simulink model "AFC_FFNN_trainlm_45_45_45_Nor_July_15"  (R2021a)
settings: Solver=ode15s  StartTime=0.0  StopTime=T  MaxStep=.01  RelTol=1e-3
undefined symbols (not defined in the file): AF_sensor_tol, fault_time, fuel_inj_tol, kappa_tol, MAF_sensor_tol, pump_tol, tau_ww_tol, x_gain, x_offset, y_gain, y_offset
libraries: neural x140
(part 1 of 6)
Description:
  | Modeling Engine Timing Using Triggered Subsystems
  | 
  | This example presents a model of a four-cylinder spark ignition engine
  | and demonstrates Simulink(R) capabilities to model an internal combustion
  | engine from the throttle to the crankshaft output. We used well-defined
  | physical principles supplemented, where appropriate, with empirical
  | relationships that describe the systems dynamic behavior without
  | introducing unnecessary complexity.
settings Model: SimulationMode=accelerator  ExtModeTrigMode=oneshot  ExtModeArmWhenConnect=off  ExtModeAutoUpdateStatusClock=off  Creator=The MathWorks Inc.  LastModifiedBy=deyun
settings SolverCC: ZeroCrossControl=DisableAll  AlgebraicLoopSolver=TrustRegion
settings DataIOCC: ExternalInput=[t__, u__]  LoadExternalInput=on  SaveFormat=StructureWithTime  SignalLogging=off  DSMLogging=off  ReturnWorkspaceOutputs=off
settings OptimizationCC: BlockReduction=off  BooleanDataType=off  LifeSpan=inf
settings DebuggingCC: SaveWithParameterizedLinksMsg=none  UnderspecifiedInitializationDetection=Classic  MergeDetectMultiDrivingBlocksExec=none  SignalResolutionControl=TryResolveAllWithWarning  ParameterPrecisionLossMsg=none  SFUnexpectedBacktrackingDiag=warning  SFNoUnconditionalDefaultTransitionDiag=warning  SFExecutionAtInitializationDiag=none  ArithmeticOperatorsInVariantConditions=warning
settings HardwareCC: ProdBitPerPointer=32  ProdBitPerSizeT=32  ProdBitPerPtrDiffT=32  ProdLargestAtomicFloat=None  ProdIntDivRoundTo=Undefined  ProdEndianess=Unspecified  ProdWordSize=32  ProdHWDeviceType=32-bit Generic  TargetBitPerLong=64  TargetBitPerPointer=64  TargetBitPerSizeT=64  TargetBitPerPtrDiffT=64  TargetLongLongMode=on  TargetIntDivRoundTo=Zero  TargetEndianess=LittleEndian  TargetWordSize=64  TargetHWDeviceType=MATLAB Host  ProdEqTarget=off
settings ModelReferenceCC: PropagateSignalLabelsOutOfModel=off
settings SFSimCC: SimUseLocalCustomCode=off  CustomCodeUndefinedFunction=UseInterfaceOnly
settings RTWCC: RTWUseLocalCustomCode=off
settings CodeAppCC: StateflowObjectComments=on
settings GRTTargetCC: TargetLangStandard=C89/C90 (ANSI)
settings ConfigComp: CovMetricSettings=d  CovSaveCumulativeToWorkspaceVar=on  CovSaveSingleToWorkspaceVar=on  CovExternalEMLEnable=off  CovBoundaryAbsTol=1.0e-5

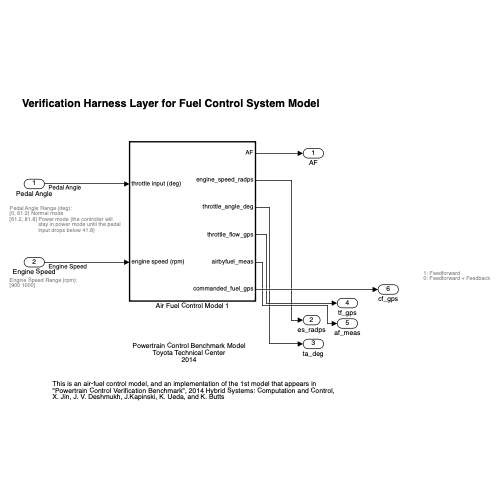
[thumbnail: Simulink's stored preview of the top-level diagram]
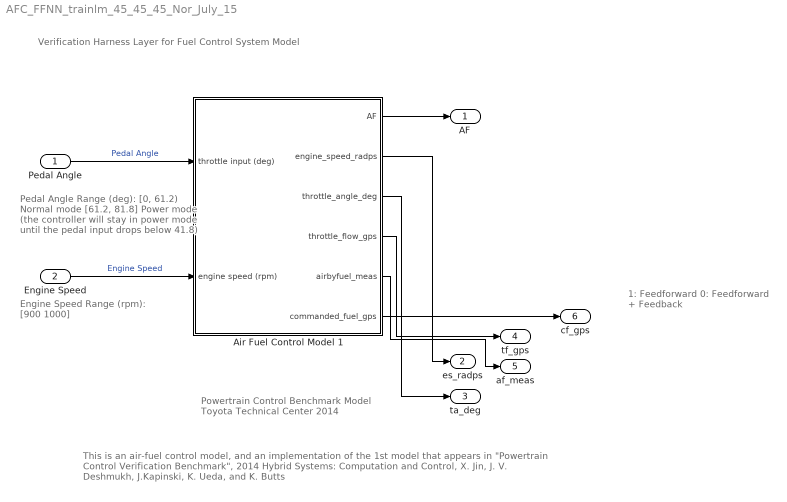
== system AFC_FFNN_trainlm_45_45_45_Nor_July_15 ==
  note: 1: Feedforward
      | 0: Feedforward + Feedback
  note: Pedal Angle Range (deg):
      | [0, 61.2) Normal mode
      | [61.2, 81.8] Power mode (the controller will
      |                    stay in power mode until the pedal
      |                    input drops below 41.8)
  note: This is an air-fuel control model, and an implementation of the 1st model that appears in
      | "Powertrain Control Verification Benchmark", 2014 Hybrid Systems: Computation and Control,
      | X. Jin, J. V. Deshmukh, J.Kapinski, K. Ueda, and K. Butts
  note: Engine Speed Range (rpm):
      | [900 1000]
  note: Powertrain Control Benchmark Model
      | Toyota Technical Center
      | 2014
  note: Verification Harness Layer for Fuel Control System Model
  Pedal Angle : Inport  Interpolate=off
  Engine Speed : Inport  Port=2  Interpolate=off
  Air Fuel Control Model 1 : Subsystem  Priority=1  TreatAsAtomicUnit=on
  AF : Outport  VectorParamsAs1DForOutWhenUnconnected=off
  es_radps : Outport  Port=2
  ta_deg : Outport  Port=3
  tf_gps : Outport  Port=4
  af_meas : Outport  Port=5
  cf_gps : Outport  Port=6
  wires:
  Air Fuel Control Model 1/1(AF) -> AF/1
  Pedal Angle/1 -> Air Fuel Control Model 1/1(throttle input (deg))  "Pedal Angle"
  Engine Speed/1 -> Air Fuel Control Model 1/2(engine speed (rpm))  "Engine Speed"
  Air Fuel Control Model 1/2(engine_speed_radps) -> es_radps/1
  Air Fuel Control Model 1/3(throttle_angle_deg) -> ta_deg/1
  Air Fuel Control Model 1/4(throttle_flow_gps) -> tf_gps/1
  Air Fuel Control Model 1/5(airbyfuel_meas) -> af_meas/1
  Air Fuel Control Model 1/6(commanded_fuel_gps) -> cf_gps/1

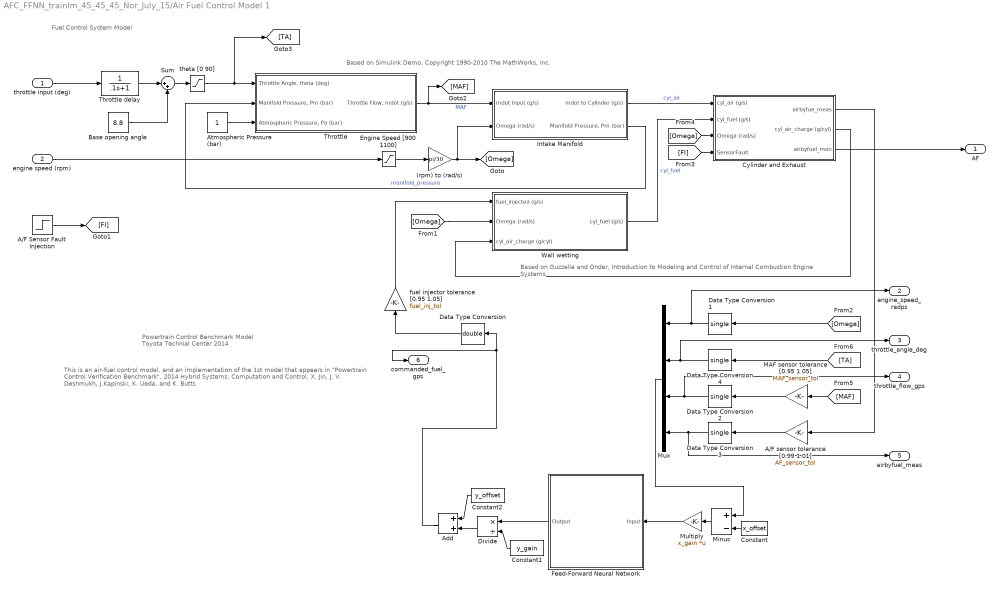
== system AFC_FFNN_trainlm_45_45_45_Nor_July_15/Air Fuel Control Model 1 ==
  note: Based on Simulink Demo, Copyright 1990-2010 The MathWorks, Inc.
  note: Based on Guzzella and Onder, Introduction to Modeling and Control of Internal Combustion Engine Systems
  note: Fuel Control System Model
  note: This is an air-fuel control model, and an implementation of the 1st model that appears in
      | "Powertrain Control Verification Benchmark", 2014 Hybrid Systems: Computation and Control,
      | X. Jin, J. V. Deshmukh, J.Kapinski, K. Ueda, and K. Butts
  note: Powertrain Control Benchmark Model
      | Toyota Technial Center
      | 2014
  throttle input (deg) : Inport  Description=[0, 81.2]
      settings: AttributesFormatString=%<Description>
  engine speed (rpm) : Inport  Description=[900,1100]  Port=2
      settings: AttributesFormatString=%<Description>
  (rpm) to (rad/s) : Gain  Gain=pi/30
  A/F Sensor Fault Injection : Step  Time=fault_time  SampleTime=0
      settings: AttributesFormatString=1: Failure\n0: Normal
  A/F sensor tolerance [0.99 1.01] : Gain  Gain=AF_sensor_tol
  Add : Sum
  Atmospheric Pressure (bar) : Constant
  Base opening angle : Constant  Value=8.8
  Constant : Constant  Value=x_offset
  Constant1 : Constant  Value=y_gain
  Constant2 : Constant  Value=y_offset
  Cylinder and Exhaust : Subsystem
  Data Type Conversion : DataTypeConversion  OutDataTypeStr=double
  Data Type Conversion{1..4} (4 alike) : DataTypeConversion  OutDataTypeStr=single
  Divide : Product  Inputs=*/
  Engine Speed [900 1100] : Saturate  UpperLimit=1100  LowerLimit=900
  Feed-Forward Neural Network : Subsystem
      mask help: Feed-Forward Neural Network
      mask Display: e = 0.06;c1 = [120 150 230]/255;c2 = ([120 150 230]+0)/383;c3 = ([120 150 230]+128)/383;patch([0 1 1 0],[0 0 1 1],c1);patch([0 1 1 1-e 1-e 0+e],[0 0 1 1-e 0+e 0+e],c2);patch([0 0 1 1-e 0+e 0+e],[0 1 1 1-e 1-e 0+e],c3);plot([0 1 1 0 0],[0 0 1 1 0]);fprintf('NNET');port_label('input',1,' Input');port_label('output',1,'Output ');
  Intake Manifold : Subsystem
  MAF sensor tolerance [0.95 1.05] : Gain  Gain=MAF_sensor_tol
  Minus : Sum  Inputs=+-
  Multiply : Gain  Gain=x_gain  Multiplication=Matrix(K*u)
  Mux : Mux
  Sum : Sum  Inputs=|++
  Throttle : Subsystem
  Throttle delay : TransferFcn  Denominator=[.1 1]
  Wall wetting : Subsystem
  fuel injector tolerance [0.95 1.05] : Gain  Gain=fuel_inj_tol
  theta [0 90] : Saturate  UpperLimit=90  LowerLimit=0
  AF : Outport  VectorParamsAs1DForOutWhenUnconnected=off
  engine_speed_radps : Outport  Port=2
  throttle_angle_deg : Outport  Port=3
  throttle_flow_gps : Outport  Port=4
  airbyfuel_meas : Outport  Port=5
  commanded_fuel_gps : Outport  Port=6
  wires:
  (rpm) to (rad/s)/1 -> [Omega], Intake Manifold/2(Omega (rad/s))
  Data Type Conversion/1 -> fuel injector tolerance [0.95 1.05]/1
  theta [0 90]/1 -> Throttle/1("Throttle Angle, theta (deg)"), [TA]
  Engine Speed [900 1100]/1 -> (rpm) to (rad/s)/1
  Cylinder and Exhaust/3("airbyfuel_mon ") -> AF/1
  A/F sensor tolerance [0.99 1.01]/1 -> Data Type Conversion3/1
  [MAF] -> MAF sensor tolerance [0.95 1.05]/1
  Cylinder and Exhaust/1(airbyfue_meas) -> A/F sensor tolerance [0.99 1.01]/1
  Throttle/1("Throttle Flow, mdot (g/s)") -> [MAF], Intake Manifold/1(mdot Input (g/s))  "MAF"
  Intake Manifold/2("Manifold Pressure, Pm (bar)") -> Throttle/2("Manifold Pressure, Pm (bar)")  "manifold_pressure"
  Atmospheric Pressure (bar)/1 -> Throttle/3("Atmospheric Pressure, Pa (bar) ")
  Wall wetting/1(cyl_fuel (g/s)) -> Cylinder and Exhaust/2(cyl_fuel (g/s))  "cyl_fuel"
  Intake Manifold/1(mdot to Cylinder (g/s)) -> Cylinder and Exhaust/1(cyl_air (g/s))  "cyl_air"
  [Omega] -> Cylinder and Exhaust/3(Omega (rad/s))
  [Omega] -> Wall wetting/2(Omega (rad/s))
  Cylinder and Exhaust/2(cyl_air_charge (g/cyl)) -> Wall wetting/3(cyl_air_charge (g/cyl))
  [Omega] -> Data Type Conversion1/1
  fuel injector tolerance [0.95 1.05]/1 -> Wall wetting/1(fuel_injected (g/s))
  MAF sensor tolerance [0.95 1.05]/1 -> Data Type Conversion2/1
  Add/1 -> Data Type Conversion/1, commanded_fuel_gps/1
  A/F Sensor Fault Injection/1 -> [FI]
  [FI] -> Cylinder and Exhaust/4(SensorFault)
  [TA] -> Data Type Conversion4/1
  throttle input (deg)/1 -> Throttle delay/1
  engine speed (rpm)/1 -> Engine Speed [900 1100]/1
  Throttle delay/1 -> Sum/1
  Base opening angle/1 -> Sum/2
  Sum/1 -> theta [0 90]/1
  Data Type Conversion3/1 -> airbyfuel_meas/1, Mux/4
  Data Type Conversion4/1 -> Mux/2, throttle_angle_deg/1
  Data Type Conversion2/1 -> Mux/3, throttle_flow_gps/1
  Data Type Conversion1/1 -> Mux/1, engine_speed_radps/1
  Multiply/1 -> Feed-Forward Neural Network/1(Input)
  Constant/1 -> Minus/2
  Mux/1 -> Minus/1
  Minus/1 -> Multiply/1
  Constant2/1 -> Add/1
  Feed-Forward Neural Network/1(Output) -> Divide/1
  Constant1/1 -> Divide/2
  Divide/1 -> Add/2

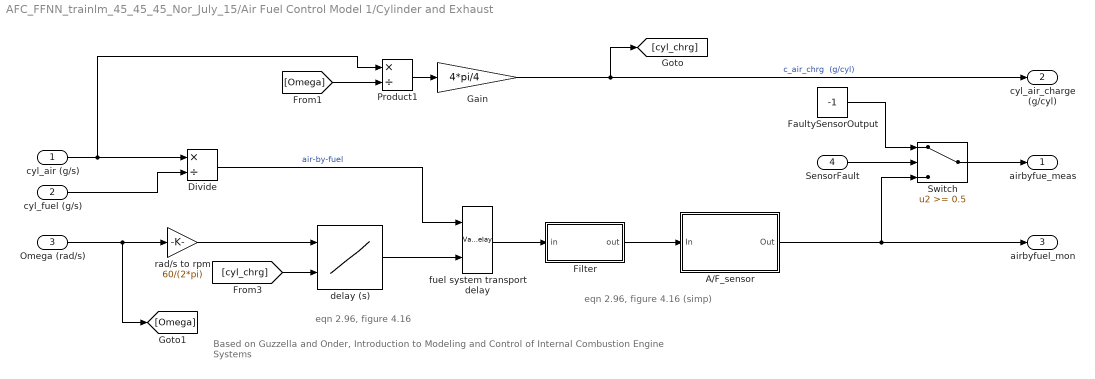
== system AFC_FFNN_trainlm_45_45_45_Nor_July_15/Air Fuel Control Model 1/Cylinder and Exhaust ==
  note: Based on Guzzella and Onder, Introduction to Modeling and Control of Internal Combustion Engine Systems
  note: eqn 2.96, figure 4.16
  note: eqn 2.96, figure 4.16 (simp)
  cyl_air (g/s) : Inport
  cyl_fuel (g/s) : Inport  Port=2
  Omega (rad/s) : Inport  Port=3
  SensorFault : Inport  Port=4
  A/F_sensor : Subsystem
  Divide : Product  Inputs=*/
  FaultySensorOutput : Constant  Value=-1
  Filter : Subsystem
  Gain : Gain  Gain=4*pi/4
  Product1 : Product  Inputs=*/  RndMeth=Zero
  Switch : Switch  Threshold=0.5
  delay (s) : Lookup_n-D  BreakpointsForDimension1=[800,1000,1500,2000,3000]  BreakpointsForDimension2=[0.05,0.15,0.2,0.25]  Table=reshape([0.8,0.6,0.4,0.3,0.2,0.4,0.3,0.2,0.2,0.2,0.3,0.25,0.2,0.2,0.2,0.25,0.2,0.2,0.2,0.2],5,4)  UseLastTableValue=on  RndMeth=Simplest  InputSameDT=on
      settings: InputPortMap=u0,u1
  fuel system transport delay : VariableTransportDelay  VariableDelayType=Variable transport delay  MaximumDelay=10  InitialOutput=14.7  MaximumPoints=20480
  rad/s to rpm : Gain  Gain=60/(2*pi)
  airbyfue_meas : Outport  VectorParamsAs1DForOutWhenUnconnected=off
  cyl_air_charge (g/cyl) : Outport  Port=2  VectorParamsAs1DForOutWhenUnconnected=off
  "airbyfuel_mon " : Outport  Port=3  VectorParamsAs1DForOutWhenUnconnected=off
  wires:
  cyl_air (g/s)/1 -> Divide/1, Product1/1
  [Omega] -> Product1/2
  Product1/1 -> Gain/1
  Gain/1 -> [cyl_chrg], cyl_air_charge (g/cyl)/1  "c_air_chrg  (g/cyl)"
  [cyl_chrg] -> delay (s)/2
  cyl_fuel (g/s)/1 -> Divide/2
  Omega (rad/s)/1 -> [Omega], rad/s to rpm/1
  rad/s to rpm/1 -> delay (s)/1
  delay (s)/1 -> fuel system transport delay/2
  fuel system transport delay/1 -> Filter/1(in)
  Switch/1 -> airbyfue_meas/1
  Divide/1 -> fuel system transport delay/1  "air-by-fuel"
  Filter/1(out) -> A/F_sensor/1(In)
  FaultySensorOutput/1 -> Switch/1
  SensorFault/1 -> Switch/2
  A/F_sensor/1(Out) -> Switch/3, "airbyfuel_mon "/1

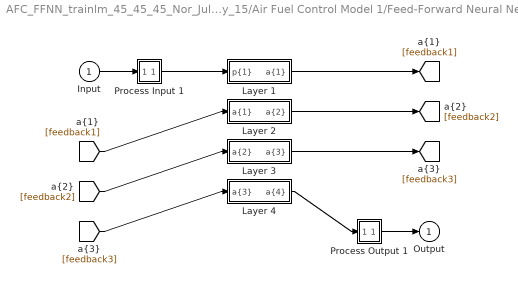
== system AFC_FFNN_trainlm_45_45_45_Nor_July_15/Air Fuel Control Model 1/Feed-Forward Neural Network ==
  Input : Inport  PortDimensions=4
      mask Display: e = 0.06;c1 = [120 230 180]/255;c2 = ([120 230 180]+0)/(256+128);c3 = ([120 230 180]+128)/(256+128);patch([0 1 1 0],[0 0 1 1],c1);patch([0 1 1 1-e 1-e 0+e],[0 0 1 1-e 0+e 0+e],c2);patch([0 0 1 1-e 0+e 0+e],[0 1 1 1-e 1-e 0+e],c3);plot([0 1 1 0 0],[0 0 1 1 0]);
  Layer 1 : Subsystem
      mask Display: e = 0.06;c1 = [120 150 230]/255;c2 = ([120 150 230]+0)/383;c3 = ([120 150 230]+128)/383;patch([0 1 1 0],[0 0 1 1],c1);patch([0 1 1 1-e 1-e 0+e],[0 0 1 1-e 0+e 0+e],c2);patch([0 0 1 1-e 0+e 0+e],[0 1 1 1-e 1-e 0+e],c3);plot([0 1 1 0 0],[0 0 1 1 0]);
  Layer 2 : Subsystem
      mask Display: e = 0.06;c1 = [120 150 230]/255;c2 = ([120 150 230]+0)/383;c3 = ([120 150 230]+128)/383;patch([0 1 1 0],[0 0 1 1],c1);patch([0 1 1 1-e 1-e 0+e],[0 0 1 1-e 0+e 0+e],c2);patch([0 0 1 1-e 0+e 0+e],[0 1 1 1-e 1-e 0+e],c3);plot([0 1 1 0 0],[0 0 1 1 0]);
  Layer 3 : Subsystem
      mask Display: e = 0.06;c1 = [120 150 230]/255;c2 = ([120 150 230]+0)/383;c3 = ([120 150 230]+128)/383;patch([0 1 1 0],[0 0 1 1],c1);patch([0 1 1 1-e 1-e 0+e],[0 0 1 1-e 0+e 0+e],c2);patch([0 0 1 1-e 0+e 0+e],[0 1 1 1-e 1-e 0+e],c3);plot([0 1 1 0 0],[0 0 1 1 0]);
  Layer 4 : Subsystem
      mask Display: e = 0.06;c1 = [120 150 230]/255;c2 = ([120 150 230]+0)/383;c3 = ([120 150 230]+128)/383;patch([0 1 1 0],[0 0 1 1],c1);patch([0 1 1 1-e 1-e 0+e],[0 0 1 1-e 0+e 0+e],c2);patch([0 0 1 1-e 0+e 0+e],[0 1 1 1-e 1-e 0+e],c3);plot([0 1 1 0 0],[0 0 1 1 0]);
  Process Input 1 : Subsystem
      mask Display: e = 0.06;c1 = [120 150 230]/255;c2 = ([120 150 230]+0)/383;c3 = ([120 150 230]+128)/383;patch([0 1 1 0],[0 0 1 1],c1);patch([0 1 1 1-e 1-e 0+e],[0 0 1 1-e 0+e 0+e],c2);patch([0 0 1 1-e 0+e 0+e],[0 1 1 1-e 1-e 0+e],c3);plot([0 1 1 0 0],[0 0 1 1 0]);
  Process Output 1 : Subsystem
      mask Display: e = 0.06;c1 = [120 150 230]/255;c2 = ([120 150 230]+0)/383;c3 = ([120 150 230]+128)/383;patch([0 1 1 0],[0 0 1 1],c1);patch([0 1 1 1-e 1-e 0+e],[0 0 1 1-e 0+e 0+e],c2);patch([0 0 1 1-e 0+e 0+e],[0 1 1 1-e 1-e 0+e],c3);plot([0 1 1 0 0],[0 0 1 1 0]);
  Output : Outport  InitialOutput=0
      mask Display: e = 0.06;c1 = [120 230 180]/255;c2 = ([120 230 180]+0)/(256+128);c3 = ([120 230 180]+128)/(256+128);patch([0 1 1 0],[0 0 1 1],c1);patch([0 1 1 1-e 1-e 0+e],[0 0 1 1-e 0+e 0+e],c2);patch([0 0 1 1-e 0+e 0+e],[0 1 1 1-e 1-e 0+e],c3);plot([0 1 1 0 0],[0 0 1 1 0]);
  wires:
  Layer 4/1("a{4}") -> Process Output 1/1(a)
  [feedback3] -> Layer 4/1("a{3} ")
  Layer 3/1("a{3}") -> [feedback3]
  [feedback2] -> Layer 3/1("a{2} ")
  Layer 2/1("a{2}") -> [feedback2]
  [feedback1] -> Layer 2/1("a{1} ")
  Layer 1/1("a{1}") -> [feedback1]
  Process Input 1/1(p) -> Layer 1/1("p{1}")
  Process Output 1/1(y) -> Output/1
  Input/1 -> Process Input 1/1(x)

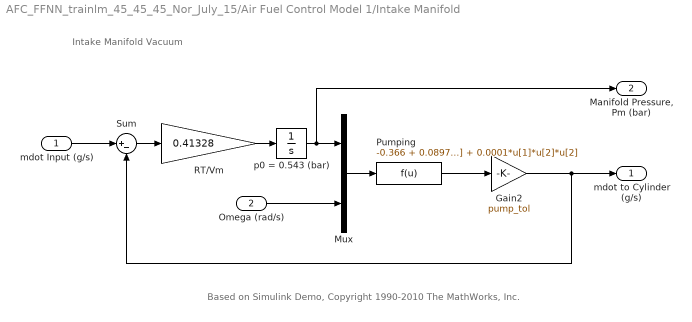
== system AFC_FFNN_trainlm_45_45_45_Nor_July_15/Air Fuel Control Model 1/Intake Manifold ==
  note: Intake Manifold Vacuum
  note: Based on Simulink Demo, Copyright 1990-2010 The MathWorks, Inc.
  mdot Input (g/s) : Inport
  Omega (rad/s) : Inport  Port=2
  Gain2 : Gain  Gain=pump_tol  ParamDataTypeStr=single  OutDataTypeStr=Inherit: Inherit via back propagation  RndMeth=Simplest  SaturateOnIntegerOverflow=on
      settings: AttributesFormatString=pumping tolerance [0.9 1.1]
  Mux : Mux  Inputs=2
  Pumping : Fcn  Expr=-0.366 + 0.08979*u[1]*u[2] - 0.0337*u[2]*u[1]*u[1] + 0.0001*u[1]*u[2]*u[2]
  RT/Vm : Gain  Gain=0.41328  SaturateOnIntegerOverflow=on  OutDataTypeStr=Inherit: Same as input  ParamDataTypeStr=Inherit: Same as input
  Sum : Sum  Inputs=|+-  InputSameDT=on  SaturateOnIntegerOverflow=on  OutDataTypeStr=Inherit: Same as first input
  p0 = 0.543 (bar) : Integrator  InitialCondition=0.982
  mdot to Cylinder (g/s) : Outport  InitialOutput=0  VectorParamsAs1DForOutWhenUnconnected=off
  "Manifold Pressure, Pm (bar)" : Outport  Port=2  InitialOutput=0  VectorParamsAs1DForOutWhenUnconnected=off
  wires:
  mdot Input (g/s)/1 -> Sum/1
  RT/Vm/1 -> p0 = 0.543 (bar)/1
  Omega (rad/s)/1 -> Mux/2
  Mux/1 -> Pumping/1
  p0 = 0.543 (bar)/1 -> Mux/1, "Manifold Pressure, Pm (bar)"/1
  Sum/1 -> RT/Vm/1
  Pumping/1 -> Gain2/1
  Gain2/1 -> Sum/2, mdot to Cylinder (g/s)/1

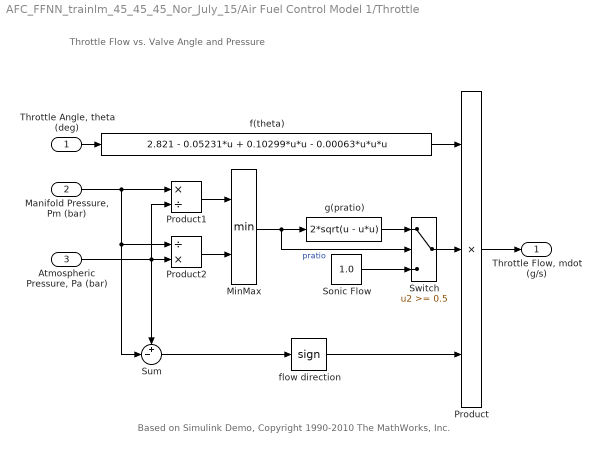
== system AFC_FFNN_trainlm_45_45_45_Nor_July_15/Air Fuel Control Model 1/Throttle ==
  note: Throttle Flow vs. Valve Angle and Pressure
  note: Based on Simulink Demo, Copyright 1990-2010 The MathWorks, Inc.
  "Throttle Angle, theta (deg)" : Inport
  "Manifold Pressure, Pm (bar)" : Inport  Port=2
  "Atmospheric Pressure, Pa (bar) " : Inport  Port=3
  MinMax : MinMax  Inputs=2  InputSameDT=on  SaturateOnIntegerOverflow=on
  Product : Product  Inputs=3  InputSameDT=on  RndMeth=Zero  SaturateOnIntegerOverflow=on  OutDataTypeStr=Inherit: Same as first input
  Product1 : Product  Inputs=*/  InputSameDT=on  RndMeth=Zero  SaturateOnIntegerOverflow=on  OutDataTypeStr=Inherit: Same as first input
  Product2 : Product  Inputs=/*  InputSameDT=on  RndMeth=Zero  SaturateOnIntegerOverflow=on  OutDataTypeStr=Inherit: Same as first input
  "Sonic Flow " : Constant  Value=1.0
  Sum : Sum  Inputs=+-|  InputSameDT=on  SaturateOnIntegerOverflow=on  OutDataTypeStr=Inherit: Same as first input
  Switch : Switch  Threshold=0.5  SaturateOnIntegerOverflow=on  InputSameDT=on
  f(theta) : Fcn  Expr=2.821 - 0.05231*u + 0.10299*u*u - 0.00063*u*u*u
  flow direction : Signum
  g(pratio) : Fcn  Expr=2*sqrt(u - u*u)
  "Throttle Flow, mdot (g/s)" : Outport  InitialOutput=0  VectorParamsAs1DForOutWhenUnconnected=off
  wires:
  "Manifold Pressure, Pm (bar)"/1 -> Sum/2, Product2/1, Product1/1
  Product2/1 -> MinMax/2
  Product1/1 -> MinMax/1
  "Atmospheric Pressure, Pa (bar) "/1 -> Sum/1, Product2/2, Product1/2
  g(pratio)/1 -> Switch/1
  "Sonic Flow "/1 -> Switch/3
  Switch/1 -> Product/2
  flow direction/1 -> Product/3
  Sum/1 -> flow direction/1
  MinMax/1 -> g(pratio)/1, Switch/2  "pratio"
  "Throttle Angle, theta (deg)"/1 -> f(theta)/1
  Product/1 -> "Throttle Flow, mdot (g/s)"/1
  f(theta)/1 -> Product/1

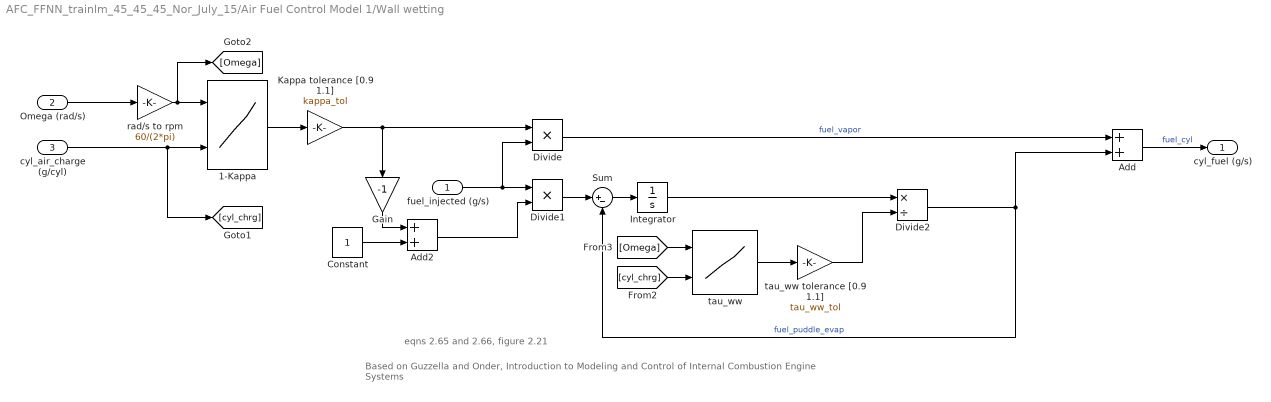
== system AFC_FFNN_trainlm_45_45_45_Nor_July_15/Air Fuel Control Model 1/Wall wetting ==
  note: Based on Guzzella and Onder, Introduction to Modeling and Control of Internal Combustion Engine Systems
  note: eqns 2.65 and 2.66, figure 2.21
  fuel_injected (g/s) : Inport
  Omega (rad/s) : Inport  Port=2
  cyl_air_charge (g/cyl) : Inport  Port=3
  1-Kappa : Lookup_n-D  BreakpointsForDimension1=[1000,1500,2000,2500,3000]  BreakpointsForDimension2=[.1,.2,.3,.4]  Table=reshape([0.8,.7,.7,.8,.9,.7,.66,.65,.73,.85,.66,.66,.63,.66,.8,.6,.6,.6,.6,.7],5,4)  UseLastTableValue=on  RndMeth=Simplest  InputSameDT=on
      settings: InputPortMap=u0,u1
  Add : Sum
  Add2 : Sum
  Constant : Constant
  Divide : Product  Inputs=**
  Divide1 : Product  Inputs=**
  Divide2 : Product  Inputs=*/
  Gain : Gain  Gain=-1
  Integrator : Integrator  InitialCondition=.0112
  Kappa tolerance [0.9 1.1] : Gain  Gain=kappa_tol
  Sum : Sum  Inputs=|+-
  rad/s to rpm : Gain  Gain=60/(2*pi)
  tau_ww : Lookup_n-D  BreakpointsForDimension1=[1000,1500,2000,2500,3000]  BreakpointsForDimension2=[0.1,0.2,0.3,0.4]  Table=reshape([.4,.3,.35,.3,.2,.22,.22,.4,.35,.5,.20,.22,.5,.4,.35,.35,.3,.45,.5,.4],5,4)  UseLastTableValue=on  RndMeth=Simplest  InputSameDT=on
      settings: InputPortMap=u0,u1
  tau_ww tolerance [0.9 1.1] : Gain  Gain=tau_ww_tol
  cyl_fuel (g/s) : Outport  VectorParamsAs1DForOutWhenUnconnected=off
  wires:
  1-Kappa/1 -> Kappa tolerance [0.9 1.1]/1
  fuel_injected (g/s)/1 -> Divide/2, Divide1/1
  Divide/1 -> Add/1  "fuel_vapor"
  Add/1 -> cyl_fuel (g/s)/1  "fuel_cyl"
  Integrator/1 -> Divide2/1
  Divide1/1 -> Sum/1
  Sum/1 -> Integrator/1
  Divide2/1 -> Add/2, Sum/2  "fuel_puddle_evap"
  Add2/1 -> Divide1/2
  cyl_air_charge (g/cyl)/1 -> 1-Kappa/2, [cyl_chrg]
  [cyl_chrg] -> tau_ww/2
  tau_ww/1 -> tau_ww tolerance [0.9 1.1]/1
  Gain/1 -> Add2/1
  Constant/1 -> Add2/2
  rad/s to rpm/1 -> [Omega], 1-Kappa/1
  Omega (rad/s)/1 -> rad/s to rpm/1
  Kappa tolerance [0.9 1.1]/1 -> Divide/1, Gain/1
  tau_ww tolerance [0.9 1.1]/1 -> Divide2/2
  [Omega] -> tau_ww/1

== system AFC_FFNN_trainlm_45_45_45_Nor_July_15/Air Fuel Control Model 1/Cylinder and Exhaust/A//F_sensor ==
  In : Inport
  A/F_sensor : Gain  OutDataTypeStr=double
  Filter : Subsystem
  Out : Outport  VectorParamsAs1DForOutWhenUnconnected=off
  wires:
  A/F_sensor/1 -> Out/1
  In/1 -> Filter/1(In)
  Filter/1(Out) -> A/F_sensor/1

== system AFC_FFNN_trainlm_45_45_45_Nor_July_15/Air Fuel Control Model 1/Cylinder and Exhaust/Filter ==
  in : Inport
  Gain1 : Gain  Gain=10
  Integrator : Integrator  InitialCondition=14.7
  Sum : Sum  Inputs=|+-
  out : Outport  VectorParamsAs1DForOutWhenUnconnected=off
  wires:
  Integrator/1 -> out/1, Sum/2
  in/1 -> Sum/1
  Gain1/1 -> Integrator/1
  Sum/1 -> Gain1/1

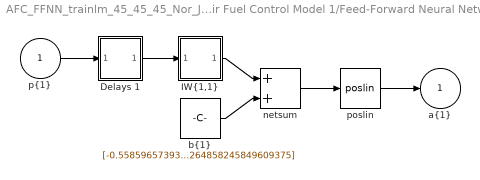
== system AFC_FFNN_trainlm_45_45_45_Nor_July_15/Air Fuel Control Model 1/Feed-Forward Neural Network/Layer 1 ==
  "p{1}" : Inport  PortDimensions=4
      mask Display: e = 0.06;c1 = [120 230 180]/255;c2 = ([120 230 180]+0)/(256+128);c3 = ([120 230 180]+128)/(256+128);patch([0 1 1 0],[0 0 1 1],c1);patch([0 1 1 1-e 1-e 0+e],[0 0 1 1-e 0+e 0+e],c2);patch([0 0 1 1-e 0+e 0+e],[0 1 1 1-e 1-e 0+e],c3);plot([0 1 1 0 0],[0 0 1 1 0]);
  Delays 1 : Subsystem
      mask Display: e = 0.06;c1 = [120 150 230]/255;c2 = ([120 150 230]+0)/383;c3 = ([120 150 230]+128)/383;patch([0 1 1 0],[0 0 1 1],c1);patch([0 1 1 1-e 1-e 0+e],[0 0 1 1-e 0+e 0+e],c2);patch([0 0 1 1-e 0+e 0+e],[0 1 1 1-e 1-e 0+e],c3);plot([0 1 1 0 0],[0 0 1 1 0]);disp('0');
  "IW{1,1}" : Subsystem
      mask Display: e = 0.06;c1 = [120 150 230]/255;c2 = ([120 150 230]+0)/383;c3 = ([120 150 230]+128)/383;patch([0 1 1 0],[0 0 1 1],c1);patch([0 1 1 1-e 1-e 0+e],[0 0 1 1-e 0+e 0+e],c2);patch([0 0 1 1-e 0+e 0+e],[0 1 1 1-e 1-e 0+e],c3);plot([0 1 1 0 0],[0 0 1 1 0]);disp('W');
  "b{1}" : Constant  Value=[-0.5585965739320057910077821361483074724674224853515625;-0.77112950387139012065063070622272789478302001953125;0.22894666757716020111246280066552571952342987060546875;-0.305047379583083699827739110332913696765899658203125;-0.69451441467543661989481051932671107351779937744140625;0.39214635280524723359718564097420312464237213134765625;-0.1555721937487436756786252090023481287062168121337890625;0.274827394729951490770503141902736388146877288818359375;0.277365245819692296525005303919897414743900299072265625;-0.1524186026109950187201746985010686330497264862060546875;-0.0018307247949869154268753845826722681522369384765625;0.58822997451524916545650967236724682152271270751953125;0.55084837701463318371253308214363642036914825439453125;0.314130170445041712046219117837608791887760162353515625;-0.07693509824360840465562461076842737384140491485595703125;-0.851136421274869547914931899867951869964599609375;0.362298342175110754670441792768542654812335968017578125;0.21255578744349323816464902847656048834323883056640625;-0.3824877228684744334685774447279982268810272216796875;-0.6749591132024963524571603556978516280651092529296875;-0.63890547966722144312967657242552377283573150634765625;-0.149732930796697971675968119598110206425189971923828125;-0.933207190422134402751908055506646633148193359375;0.10402318613955320592001640989110455848276615142822265625;0.829936502547987675626472992007620632648468017578125;-0.737888972575629242811601216089911758899688720703125;0.21732415928306558772220569153432734310626983642578125;-0.1580532967861125737130123525275848805904388427734375;-1.288298758066100280217369800084270536899566650390625;-0.9481540190806569956549765265663154423236846923828125;0.942806016112406108931054404820315539836883544921875;-0.439159443551665196192601570146507583558559417724609375;0.276425093592411907916783775363001041114330291748046875;0.485464567417084047473707641984219662845134735107421875;0.295746825087029263645632681800634600222110748291015625;-0.8382271786519968070905406420934014022350311279296875;-0.1591390063283328881738043492077849805355072021484375;-0.7823304156725818803153060798649676144123077392578125;0.2224216466664273028630560702367802150547504425048828125;0.75721224172485557257772370576276443898677825927734375;-0.26127862544034818892413341018254868686199188232421875;0.1681522472301393289484394699684344232082366943359375;0.00998894613673773079653983586467802524566650390625;-0.6614665456480552929718896848498843610286712646484375;-0.838290046288482582070855642086826264858245849609375]
      mask Display: e = 0.06;c1 = [120 150 230]/255;c2 = ([120 150 230]+0)/383;c3 = ([120 150 230]+128)/383;patch([0 1 1 0],[0 0 1 1],c1);patch([0 1 1 1-e 1-e 0+e],[0 0 1 1-e 0+e 0+e],c2);patch([0 0 1 1-e 0+e 0+e],[0 1 1 1-e 1-e 0+e],c3);plot([0 1 1 0 0],[0 0 1 1 0]);disp('b');
  netsum : Sum  Inputs=2  InputSameDT=on  SaturateOnIntegerOverflow=on  OutDataTypeStr=Inherit: Same as first input
      mask Display: e = 0.06;c1 = [120 150 230]/255;c2 = ([120 150 230]+0)/383;c3 = ([120 150 230]+128)/383;patch([0 1 1 0],[0 0 1 1],c1);patch([0 1 1 1-e 1-e 0+e],[0 0 1 1-e 0+e 0+e],c2);patch([0 0 1 1-e 0+e 0+e],[0 1 1 1-e 1-e 0+e],c3);plot([0 1 1 0 0],[0 0 1 1 0]);disp('+');
  poslin : neural/Transfer Functions/poslin
  "a{1}" : Outport  InitialOutput=[0;0;0;0;0;0;0;0;0;0;0;0;0;0;0;0;0;0;0;0;0;0;0;0;0;0;0;0;0;0;0;0;0;0;0;0;0;0;0;0;0;0;0;0;0]
      mask Display: e = 0.06;c1 = [120 230 180]/255;c2 = ([120 230 180]+0)/(256+128);c3 = ([120 230 180]+128)/(256+128);patch([0 1 1 0],[0 0 1 1],c1);patch([0 1 1 1-e 1-e 0+e],[0 0 1 1-e 0+e 0+e],c2);patch([0 0 1 1-e 0+e 0+e],[0 1 1 1-e 1-e 0+e],c3);plot([0 1 1 0 0],[0 0 1 1 0]);
  wires:
  poslin/1 -> "a{1}"/1
  netsum/1 -> poslin/1
  "b{1}"/1 -> netsum/2
  "IW{1,1}"/1("iz{1,1}") -> netsum/1
  Delays 1/1("pd{1,1}") -> "IW{1,1}"/1("pd{1,1}")
  "p{1}"/1 -> Delays 1/1("p{1}")

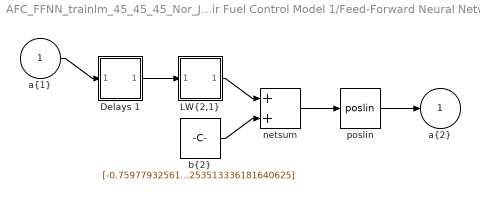
== system AFC_FFNN_trainlm_45_45_45_Nor_July_15/Air Fuel Control Model 1/Feed-Forward Neural Network/Layer 2 ==
  "a{1} " : Inport  PortDimensions=45
      mask Display: e = 0.06;c1 = [120 230 180]/255;c2 = ([120 230 180]+0)/(256+128);c3 = ([120 230 180]+128)/(256+128);patch([0 1 1 0],[0 0 1 1],c1);patch([0 1 1 1-e 1-e 0+e],[0 0 1 1-e 0+e 0+e],c2);patch([0 0 1 1-e 0+e 0+e],[0 1 1 1-e 1-e 0+e],c3);plot([0 1 1 0 0],[0 0 1 1 0]);
  Delays 1 : Subsystem
      mask Display: e = 0.06;c1 = [120 150 230]/255;c2 = ([120 150 230]+0)/383;c3 = ([120 150 230]+128)/383;patch([0 1 1 0],[0 0 1 1],c1);patch([0 1 1 1-e 1-e 0+e],[0 0 1 1-e 0+e 0+e],c2);patch([0 0 1 1-e 0+e 0+e],[0 1 1 1-e 1-e 0+e],c3);plot([0 1 1 0 0],[0 0 1 1 0]);disp('0');
  "LW{2,1}" : Subsystem
      mask Display: e = 0.06;c1 = [120 150 230]/255;c2 = ([120 150 230]+0)/383;c3 = ([120 150 230]+128)/383;patch([0 1 1 0],[0 0 1 1],c1);patch([0 1 1 1-e 1-e 0+e],[0 0 1 1-e 0+e 0+e],c2);patch([0 0 1 1-e 0+e 0+e],[0 1 1 1-e 1-e 0+e],c3);plot([0 1 1 0 0],[0 0 1 1 0]);disp('W');
  "b{2}" : Constant  Value=[-0.759779325613544553874589837505482137203216552734375;0.6965202526642186864336281360010616481304168701171875;-0.861179161880855748023577689309604465961456298828125;0.279069361418990080636604034225456416606903076171875;0.7788995695670519747721982639632187783718109130859375;0.72059847295826762181292224340722896158695220947265625;0.56823299771985691375419946780311875045299530029296875;-0.814016852489903186551600811071693897247314453125;-0.25020043213131148984729179574060253798961639404296875;0.3676809986895264170669861414353363215923309326171875;-0.5664709440966280151741329973447136580944061279296875;0.02629409189089770837455262153525836765766143798828125;-0.54936854809591240123012312324135564267635345458984375;-0.133862432529689490134927609688020311295986175537109375;-0.81332808228198449906898304107016883790493011474609375;-0.75199519420301730310285392988589592278003692626953125;-1.0530530335707963818236976294429041445255279541015625;-0.3949760005903317772180116662639193236827850341796875;0.08349711700445057449559982387654599733650684356689453125;-0.5150947870913196169340153574012219905853271484375;0.80569296901346032502289062904310412704944610595703125;-0.335455649950676171311414464071276597678661346435546875;0.2177777173381762187975851929877535440027713775634765625;-0.24227916035240870673561630610493011772632598876953125;-0.7581191909009616924919328084797598421573638916015625;-0.316127694986459373271969752750010229647159576416015625;-0.7572608648365470873642379956436343491077423095703125;-0.1771784549431406896591312261080020107328891754150390625;0.6700945036965897383396395525778643786907196044921875;-0.37793060271353240420211250238935463130474090576171875;0.49989124604212953340010017200256697833538055419921875;-0.8804292366841608430405585750122554600238800048828125;-0.68894262263308225779923077425337396562099456787109375;-0.7835754927496629829164476177538745105266571044921875;-0.331990649298899709318533268742612563073635101318359375;-0.365329678636181875983623967840685509145259857177734375;-0.1674592513076313959885510485037229955196380615234375;-0.65902586680079677794452663874835707247257232666015625;-0.045949912742535292675682967455941252410411834716796875;-0.56660135380107534697202709139673970639705657958984375;0.85478289689744979540364511194638907909393310546875;0.8907503577019373341983055070159025490283966064453125;-0.7442862631882911639280564486398361623287200927734375;0.8790617462862424513758696775767020881175994873046875;-0.487941954201235095212041414924897253513336181640625]
      mask Display: e = 0.06;c1 = [120 150 230]/255;c2 = ([120 150 230]+0)/383;c3 = ([120 150 230]+128)/383;patch([0 1 1 0],[0 0 1 1],c1);patch([0 1 1 1-e 1-e 0+e],[0 0 1 1-e 0+e 0+e],c2);patch([0 0 1 1-e 0+e 0+e],[0 1 1 1-e 1-e 0+e],c3);plot([0 1 1 0 0],[0 0 1 1 0]);disp('b');
  netsum : Sum  Inputs=2  InputSameDT=on  SaturateOnIntegerOverflow=on  OutDataTypeStr=Inherit: Same as first input
      mask Display: e = 0.06;c1 = [120 150 230]/255;c2 = ([120 150 230]+0)/383;c3 = ([120 150 230]+128)/383;patch([0 1 1 0],[0 0 1 1],c1);patch([0 1 1 1-e 1-e 0+e],[0 0 1 1-e 0+e 0+e],c2);patch([0 0 1 1-e 0+e 0+e],[0 1 1 1-e 1-e 0+e],c3);plot([0 1 1 0 0],[0 0 1 1 0]);disp('+');
  poslin : neural/Transfer Functions/poslin
  "a{2}" : Outport  InitialOutput=[0;0;0;0;0;0;0;0;0;0;0;0;0;0;0;0;0;0;0;0;0;0;0;0;0;0;0;0;0;0;0;0;0;0;0;0;0;0;0;0;0;0;0;0;0]
      mask Display: e = 0.06;c1 = [120 230 180]/255;c2 = ([120 230 180]+0)/(256+128);c3 = ([120 230 180]+128)/(256+128);patch([0 1 1 0],[0 0 1 1],c1);patch([0 1 1 1-e 1-e 0+e],[0 0 1 1-e 0+e 0+e],c2);patch([0 0 1 1-e 0+e 0+e],[0 1 1 1-e 1-e 0+e],c3);plot([0 1 1 0 0],[0 0 1 1 0]);
  wires:
  poslin/1 -> "a{2}"/1
  netsum/1 -> poslin/1
  "b{2}"/1 -> netsum/2
  "LW{2,1}"/1("lz{2,1}") -> netsum/1
  Delays 1/1("pd{2,1}") -> "LW{2,1}"/1("ad{2,1}")
  "a{1} "/1 -> Delays 1/1("p{2}")

== system AFC_FFNN_trainlm_45_45_45_Nor_July_15/Air Fuel Control Model 1/Feed-Forward Neural Network/Layer 3 ==
  "a{2} " : Inport  PortDimensions=45
      mask Display: e = 0.06;c1 = [120 230 180]/255;c2 = ([120 230 180]+0)/(256+128);c3 = ([120 230 180]+128)/(256+128);patch([0 1 1 0],[0 0 1 1],c1);patch([0 1 1 1-e 1-e 0+e],[0 0 1 1-e 0+e 0+e],c2);patch([0 0 1 1-e 0+e 0+e],[0 1 1 1-e 1-e 0+e],c3);plot([0 1 1 0 0],[0 0 1 1 0]);
  Delays 1 : Subsystem
      mask Display: e = 0.06;c1 = [120 150 230]/255;c2 = ([120 150 230]+0)/383;c3 = ([120 150 230]+128)/383;patch([0 1 1 0],[0 0 1 1],c1);patch([0 1 1 1-e 1-e 0+e],[0 0 1 1-e 0+e 0+e],c2);patch([0 0 1 1-e 0+e 0+e],[0 1 1 1-e 1-e 0+e],c3);plot([0 1 1 0 0],[0 0 1 1 0]);disp('0');
  "LW{3,2}" : Subsystem
      mask Display: e = 0.06;c1 = [120 150 230]/255;c2 = ([120 150 230]+0)/383;c3 = ([120 150 230]+128)/383;patch([0 1 1 0],[0 0 1 1],c1);patch([0 1 1 1-e 1-e 0+e],[0 0 1 1-e 0+e 0+e],c2);patch([0 0 1 1-e 0+e 0+e],[0 1 1 1-e 1-e 0+e],c3);plot([0 1 1 0 0],[0 0 1 1 0]);disp('W');
  "b{3}" : Constant  Value=[0.2734299490328331305732945111230947077274322509765625;0.253212645186324747381689803660265170037746429443359375;0.93467329178748126405906759828212670981884002685546875;0.85424049495533072029473942166077904403209686279296875;0.370732482252811246237200748510076664388179779052734375;0.58575586111893096497027499935938976705074310302734375;-0.57222729704926555971411517020897008478641510009765625;0.402075725104235726092838376644067466259002685546875;0.77510392535672212321884444463648833334445953369140625;0.89750677439359172193888980473275296390056610107421875;-0.53893848136911326474063343994203023612499237060546875;-0.447084590177655893938890585559420287609100341796875;-0.16971363346798085114386367422412149608135223388671875;-0.1253386080403514346581772542776889167726039886474609375;0.7324385856904609415352069845539517700672149658203125;-0.1718566614749994225785911794446292333304882049560546875;-0.649121257858855216227311757393181324005126953125;0.0020706443178506819292883367467084099189378321170806884765625;0.14280132148982105366741279794950969517230987548828125;-0.400326950100625911233009901479817926883697509765625;-0.09611968684726655831607189384158118627965450286865234375;-0.86780297012492602082289749887422658503055572509765625;-0.22662709591045449020185742483590729534626007080078125;-0.049925910120531102887042607108014635741710662841796875;0.957436543865733735714229624136351048946380615234375;0.557449966972769939133058869629167020320892333984375;-0.28645987977858933248853645636700093746185302734375;0.1261192693375135787103857865076861344277858734130859375;-0.5205296579813223356580920153646729886531829833984375;0.30033442526422593488177881226874887943267822265625;-0.17988670535213813206354416251997463405132293701171875;0.88536176329107918459015991174965165555477142333984375;0.52550652298814781726576939036021940410137176513671875;0.55963934687581906590736480211489833891391754150390625;0.1453135731776866723663488301099278032779693603515625;0.5122265681069091414201466250233352184295654296875;-0.3700450504693375552989209609222598373889923095703125;0.0395997938226071710676734483058680780231952667236328125;0.741921262418416826989187029539607465267181396484375;-0.1478710785470286614984303241726593114435672760009765625;0.3344458719405338786856418664683587849140167236328125;-0.562784675088596753056435773032717406749725341796875;0.6146888018342695492179927896359004080295562744140625;0.41510836491622049582161935177282430231571197509765625;0.885843136212703274878776937839575111865997314453125]
      mask Display: e = 0.06;c1 = [120 150 230]/255;c2 = ([120 150 230]+0)/383;c3 = ([120 150 230]+128)/383;patch([0 1 1 0],[0 0 1 1],c1);patch([0 1 1 1-e 1-e 0+e],[0 0 1 1-e 0+e 0+e],c2);patch([0 0 1 1-e 0+e 0+e],[0 1 1 1-e 1-e 0+e],c3);plot([0 1 1 0 0],[0 0 1 1 0]);disp('b');
  netsum : Sum  Inputs=2  InputSameDT=on  SaturateOnIntegerOverflow=on  OutDataTypeStr=Inherit: Same as first input
      mask Display: e = 0.06;c1 = [120 150 230]/255;c2 = ([120 150 230]+0)/383;c3 = ([120 150 230]+128)/383;patch([0 1 1 0],[0 0 1 1],c1);patch([0 1 1 1-e 1-e 0+e],[0 0 1 1-e 0+e 0+e],c2);patch([0 0 1 1-e 0+e 0+e],[0 1 1 1-e 1-e 0+e],c3);plot([0 1 1 0 0],[0 0 1 1 0]);disp('+');
  poslin : neural/Transfer Functions/poslin
  "a{3}" : Outport  InitialOutput=[0;0;0;0;0;0;0;0;0;0;0;0;0;0;0;0;0;0;0;0;0;0;0;0;0;0;0;0;0;0;0;0;0;0;0;0;0;0;0;0;0;0;0;0;0]
      mask Display: e = 0.06;c1 = [120 230 180]/255;c2 = ([120 230 180]+0)/(256+128);c3 = ([120 230 180]+128)/(256+128);patch([0 1 1 0],[0 0 1 1],c1);patch([0 1 1 1-e 1-e 0+e],[0 0 1 1-e 0+e 0+e],c2);patch([0 0 1 1-e 0+e 0+e],[0 1 1 1-e 1-e 0+e],c3);plot([0 1 1 0 0],[0 0 1 1 0]);
  wires:
  poslin/1 -> "a{3}"/1
  netsum/1 -> poslin/1
  "b{3}"/1 -> netsum/2
  "LW{3,2}"/1("lz{3,2}") -> netsum/1
  Delays 1/1("pd{3,2}") -> "LW{3,2}"/1("ad{3,2}")
  "a{2} "/1 -> Delays 1/1("p{3}")

== system AFC_FFNN_trainlm_45_45_45_Nor_July_15/Air Fuel Control Model 1/Feed-Forward Neural Network/Layer 4 ==
  "a{3} " : Inport  PortDimensions=45
      mask Display: e = 0.06;c1 = [120 230 180]/255;c2 = ([120 230 180]+0)/(256+128);c3 = ([120 230 180]+128)/(256+128);patch([0 1 1 0],[0 0 1 1],c1);patch([0 1 1 1-e 1-e 0+e],[0 0 1 1-e 0+e 0+e],c2);patch([0 0 1 1-e 0+e 0+e],[0 1 1 1-e 1-e 0+e],c3);plot([0 1 1 0 0],[0 0 1 1 0]);
  Delays 1 : Subsystem
      mask Display: e = 0.06;c1 = [120 150 230]/255;c2 = ([120 150 230]+0)/383;c3 = ([120 150 230]+128)/383;patch([0 1 1 0],[0 0 1 1],c1);patch([0 1 1 1-e 1-e 0+e],[0 0 1 1-e 0+e 0+e],c2);patch([0 0 1 1-e 0+e 0+e],[0 1 1 1-e 1-e 0+e],c3);plot([0 1 1 0 0],[0 0 1 1 0]);disp('0');
  "LW{4,3}" : Subsystem
      mask Display: e = 0.06;c1 = [120 150 230]/255;c2 = ([120 150 230]+0)/383;c3 = ([120 150 230]+128)/383;patch([0 1 1 0],[0 0 1 1],c1);patch([0 1 1 1-e 1-e 0+e],[0 0 1 1-e 0+e 0+e],c2);patch([0 0 1 1-e 0+e 0+e],[0 1 1 1-e 1-e 0+e],c3);plot([0 1 1 0 0],[0 0 1 1 0]);disp('W');
  "b{4}" : Constant  Value=0.2094296706820160391959717571808141656219959259033203125
      mask Display: e = 0.06;c1 = [120 150 230]/255;c2 = ([120 150 230]+0)/383;c3 = ([120 150 230]+128)/383;patch([0 1 1 0],[0 0 1 1],c1);patch([0 1 1 1-e 1-e 0+e],[0 0 1 1-e 0+e 0+e],c2);patch([0 0 1 1-e 0+e 0+e],[0 1 1 1-e 1-e 0+e],c3);plot([0 1 1 0 0],[0 0 1 1 0]);disp('b');
  netsum : Sum  Inputs=2  InputSameDT=on  SaturateOnIntegerOverflow=on  OutDataTypeStr=Inherit: Same as first input
      mask Display: e = 0.06;c1 = [120 150 230]/255;c2 = ([120 150 230]+0)/383;c3 = ([120 150 230]+128)/383;patch([0 1 1 0],[0 0 1 1],c1);patch([0 1 1 1-e 1-e 0+e],[0 0 1 1-e 0+e 0+e],c2);patch([0 0 1 1-e 0+e 0+e],[0 1 1 1-e 1-e 0+e],c3);plot([0 1 1 0 0],[0 0 1 1 0]);disp('+');
  purelin : neural/Transfer Functions/purelin
  "a{4}" : Outport  InitialOutput=0
      mask Display: e = 0.06;c1 = [120 230 180]/255;c2 = ([120 230 180]+0)/(256+128);c3 = ([120 230 180]+128)/(256+128);patch([0 1 1 0],[0 0 1 1],c1);patch([0 1 1 1-e 1-e 0+e],[0 0 1 1-e 0+e 0+e],c2);patch([0 0 1 1-e 0+e 0+e],[0 1 1 1-e 1-e 0+e],c3);plot([0 1 1 0 0],[0 0 1 1 0]);
  wires:
  purelin/1 -> "a{4}"/1
  netsum/1 -> purelin/1
  "b{4}"/1 -> netsum/2
  "LW{4,3}"/1("lz{4,3}") -> netsum/1
  Delays 1/1("pd{4,3}") -> "LW{4,3}"/1("ad{4,3}")
  "a{3} "/1 -> Delays 1/1("p{4}")

== system AFC_FFNN_trainlm_45_45_45_Nor_July_15/Air Fuel Control Model 1/Feed-Forward Neural Network/Process Input 1 ==
  x : Inport  PortDimensions=4
      mask Display: e = 0.06;c1 = [120 230 180]/255;c2 = ([120 230 180]+0)/(256+128);c3 = ([120 230 180]+128)/(256+128);patch([0 1 1 0],[0 0 1 1],c1);patch([0 1 1 1-e 1-e 0+e],[0 0 1 1-e 0+e 0+e],c2);patch([0 0 1 1-e 0+e 0+e],[0 1 1 1-e 1-e 0+e],c3);plot([0 1 1 0 0],[0 0 1 1 0]);
  p : Outport  PortDimensions=4
      mask Display: e = 0.06;c1 = [120 230 180]/255;c2 = ([120 230 180]+0)/(256+128);c3 = ([120 230 180]+128)/(256+128);patch([0 1 1 0],[0 0 1 1],c1);patch([0 1 1 1-e 1-e 0+e],[0 0 1 1-e 0+e 0+e],c2);patch([0 0 1 1-e 0+e 0+e],[0 1 1 1-e 1-e 0+e],c3);plot([0 1 1 0 0],[0 0 1 1 0]);
  wires:
  x/1 -> p/1

== system AFC_FFNN_trainlm_45_45_45_Nor_July_15/Air Fuel Control Model 1/Feed-Forward Neural Network/Process Output 1 ==
  a : Inport  PortDimensions=1
      mask Display: e = 0.06;c1 = [120 230 180]/255;c2 = ([120 230 180]+0)/(256+128);c3 = ([120 230 180]+128)/(256+128);patch([0 1 1 0],[0 0 1 1],c1);patch([0 1 1 1-e 1-e 0+e],[0 0 1 1-e 0+e 0+e],c2);patch([0 0 1 1-e 0+e 0+e],[0 1 1 1-e 1-e 0+e],c3);plot([0 1 1 0 0],[0 0 1 1 0]);
  y : Outport  PortDimensions=1
      mask Display: e = 0.06;c1 = [120 230 180]/255;c2 = ([120 230 180]+0)/(256+128);c3 = ([120 230 180]+128)/(256+128);patch([0 1 1 0],[0 0 1 1],c1);patch([0 1 1 1-e 1-e 0+e],[0 0 1 1-e 0+e 0+e],c2);patch([0 0 1 1-e 0+e 0+e],[0 1 1 1-e 1-e 0+e],c3);plot([0 1 1 0 0],[0 0 1 1 0]);
  wires:
  a/1 -> y/1

== system AFC_FFNN_trainlm_45_45_45_Nor_July_15/Air Fuel Control Model 1/Cylinder and Exhaust/A//F_sensor/Filter ==
  In : Inport
  Gain : Gain  Gain=50
  Integrator : Integrator  InitialCondition=14.7
  Sum : Sum  Inputs=|+-
  Out : Outport  VectorParamsAs1DForOutWhenUnconnected=off
  wires:
  Integrator/1 -> Out/1, Sum/2
  In/1 -> Sum/1
  Gain/1 -> Integrator/1
  Sum/1 -> Gain/1

== system AFC_FFNN_trainlm_45_45_45_Nor_July_15/Air Fuel Control Model 1/Feed-Forward Neural Network/Layer 1/Delays 1 ==
  "p{1}" : Inport  PortDimensions=4
      mask Display: e = 0.06;c1 = [120 230 180]/255;c2 = ([120 230 180]+0)/(256+128);c3 = ([120 230 180]+128)/(256+128);patch([0 1 1 0],[0 0 1 1],c1);patch([0 1 1 1-e 1-e 0+e],[0 0 1 1-e 0+e 0+e],c2);patch([0 0 1 1-e 0+e 0+e],[0 1 1 1-e 1-e 0+e],c3);plot([0 1 1 0 0],[0 0 1 1 0]);
  mux : Mux  Inputs=1
      mask Display: e = 0.06;c1 = [120 150 230]/255;c2 = ([120 150 230]+0)/383;c3 = ([120 150 230]+128)/383;patch([0 1 1 0],[0 0 1 1],c1);patch([0 1 1 1-e 1-e 0+e],[0 0 1 1-e 0+e 0+e],c2);patch([0 0 1 1-e 0+e 0+e],[0 1 1 1-e 1-e 0+e],c3);plot([0 1 1 0 0],[0 0 1 1 0]);disp('Mux')
  "pd{1,1}" : Outport
      mask Display: e = 0.06;c1 = [120 230 180]/255;c2 = ([120 230 180]+0)/(256+128);c3 = ([120 230 180]+128)/(256+128);patch([0 1 1 0],[0 0 1 1],c1);patch([0 1 1 1-e 1-e 0+e],[0 0 1 1-e 0+e 0+e],c2);patch([0 0 1 1-e 0+e 0+e],[0 1 1 1-e 1-e 0+e],c3);plot([0 1 1 0 0],[0 0 1 1 0]);
  wires:
  mux/1 -> "pd{1,1}"/1
  "p{1}"/1 -> mux/1
